simulink model "Lab2_Task_5_advanced"  (R2025b)
settings: Solver=FixedStepAuto  StartTime=0.0  StopTime=inf  RelTol=1e-3
model workspace (MAT data in the model file):
  SL_ROS_VariableLengthArrays_MaxSizes : object (value not decoded)
undefined symbols (not defined in the file or in its folder): angdiff, header, twist
libraries: ros2lib x4, simulink_extras x1, simulink x1
(part 2 of 2)

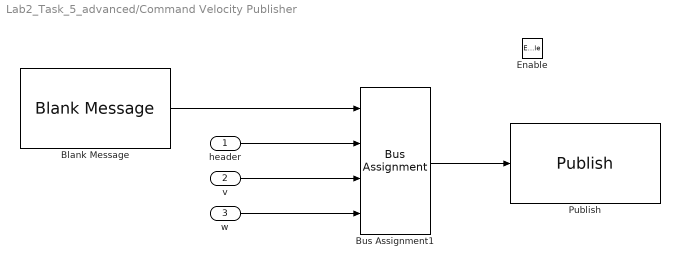
== system Lab2_Task_5_advanced/Command Velocity Publisher ==
  header : Inport
  v : Inport  Port=2
  w : Inport  Port=3
  Enable : EnablePort
  Blank Message : ros2lib/Blank Message  messageClass=Message  entityType=geometry_msgs/TwistStamped  messageType=geometry_msgs/TwistStamped  SampleTime=inf
  Bus Assignment1 : BusAssignment  DialogController=Simulink.DDGSource_BusAssignment  AssignedSignals=header,twist.linear.x,twist.angular.z
  Publish : ros2lib/Publish  topicSource=Select from ROS network  topic=/cmd_vel  messageType=geometry_msgs/TwistStamped  QOSHistory=Keep last  QOSDepth=10  QOSReliability=Reliable  QOSDurability=Volatile  QOSDeadline=Inf  QOSLifespan=Inf  QOSLiveliness=Automatic  QOSLeaseDuration=Inf  QOSAvoidROSNamespaceConventions=off
  wires:
  Bus Assignment1/1 -> Publish/1
  Blank Message/1 -> Bus Assignment1/1
  header/1 -> Bus Assignment1/2
  v/1 -> Bus Assignment1/3
  w/1 -> Bus Assignment1/4

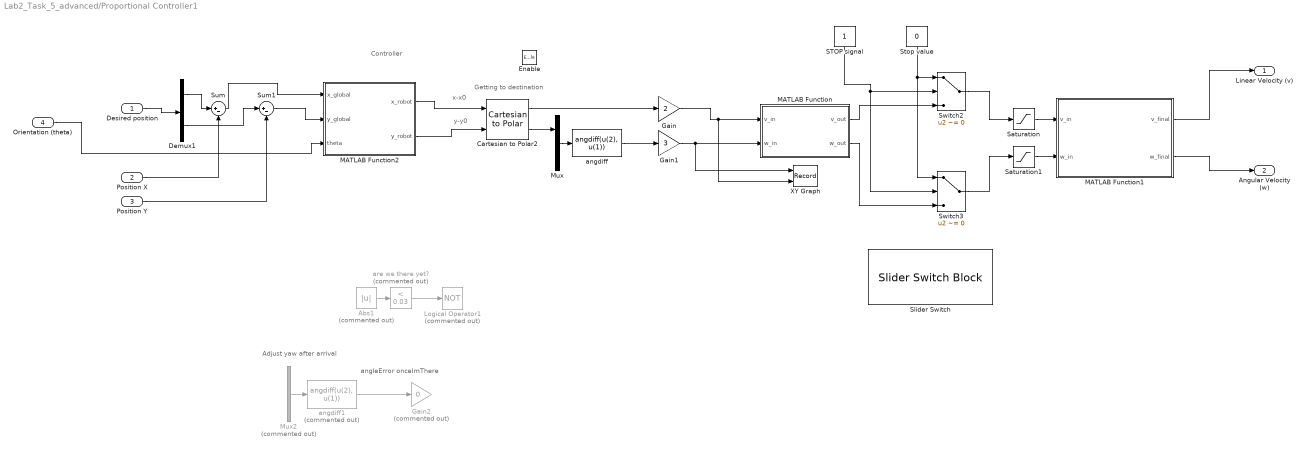
== system Lab2_Task_5_advanced/Proportional Controller1 ==
  note: angleError
      | onceImThere
  note: Controller
  note: x-x0
  note: y-y0
  note: Adjust yaw after arrival
  note: Getting to destination
  Desired position : Inport
  Position X : Inport  Port=2
  Position Y : Inport  Port=3
  Orientation (theta) : Inport  Port=4
  Enable : EnablePort
  Abs1 : Abs  Commented=on  SaturateOnIntegerOverflow=off
  Cartesian to Polar2 : simulink_extras/Transformations/Cartesian to Polar
  Demux1 : Demux  Outputs=2
  Gain : Gain  Gain=2
  Gain1 : Gain  Gain=3
  Gain2 : Gain  Commented=on  Gain=0
  Logical Operator1 : Logic  Commented=on  Operator=NOT  AllPortsSameDT=off  OutDataTypeStr=boolean
  MATLAB Function : MATLAB Function  TreatAsAtomicUnit=on
  MATLAB Function1 : MATLAB Function  TreatAsAtomicUnit=on
  MATLAB Function2 : MATLAB Function  TreatAsAtomicUnit=on
  Mux : Mux  Inputs=2
  Mux2 : Mux  Commented=on  Inputs=2
  "STOP signal " : Constant
  Saturation : Saturate  UpperLimit=0.3  LowerLimit=-0.3  LinearizeAsGain=off
  Saturation1 : Saturate  UpperLimit=999  LowerLimit=-999  LinearizeAsGain=off
  Slider Switch : SliderSwitchBlock
  Stop value : Constant  Value=0
  Sum : Sum  Inputs=|+-
  Sum1 : Sum  Inputs=|+-
  Switch2 : Switch  Criteria=u2 ~= 0  SaturateOnIntegerOverflow=off  InputSameDT=off
  Switch3 : Switch  Criteria=u2 ~= 0  SaturateOnIntegerOverflow=off  InputSameDT=off
  XY Graph : Record  NumPorts=2.0  FileSettingsInternal="{\"entries\":[{\"content\":{\"excelSettings\":{\"content\":{},\"type\":\"Streamout.ExcelSettings\"},\"parquetSettings\":{\"content\":{},\"type\":\"Streamout.ParquetSettings\"}},\"type\":\"Streamout.FileSettingStorage\",\"uuid\":\"\"}],\"packageUris\":[\"http:\\/\\/schema.mathworks.com\\/mf0\\/streamout_blocks\\/R2020a\"],\"version\":\"1.0\"}"  FrameSettings=[0, 0]  Layout=[1 1]  SignalsInternal="{\"entries\":[{\"content\":{\"signals\":[{\"content\":{\"blockPath\":[],\"dimensions\":[1],\"domain\":\"\",\"lineColor\":\"#139fff\",\"lineWidth\":2,\"port\":1,\"sid\":[\"\"],\"signalID\":1,\"signalName\":\"Gain1\"},\"type\":\"RecordBlkView.Signal\",\"uuid\":\"\"},{\"content\":{\"blockPath\":[],\"dimensions\":[1],\"domain\":\"\",\"lineColor\":\"#ff6929\",\"lineWidth\":2,\"port\":2,\"sid\":[\"\"],\"signalID\":2,\"signalName\":\"Gain\"},\"type\":\"RecordBlkView.Signal\",\"uuid\":\"\"}]},\"type\":\"RecordBlkView.InputSignals\",\"uuid\":\"\"}],\"packageUris\":[\"http:\\/\\/schema.mathworks.com\\/mf0\\/streamout_blocks\\/R2020a\"],\"version\":\"1.0\"}"  VisualizationBindings="{\"xyplotplugin\":{\"info\":[{\"series\":[],\"subplotID\":1}]}}"  CompatibilityTag=XY
  angdiff : MATLABFcn  MATLABFcn=angdiff(u(2), u(1))  OutputDimensions=1  Output1D=off
  angdiff1 : MATLABFcn  Commented=on  MATLABFcn=angdiff(u(2), u(1))  OutputDimensions=1  Output1D=off
  are we there yet? : simulink/Logic and Bit Operations/Compare To Constant  Commented=on  relop=<  const=0.03  OutDataTypeStr=boolean
  Linear Velocity (v) : Outport  VectorParamsAs1DForOutWhenUnconnected=off
  Angular Velocity (w) : Outport  Port=2  VectorParamsAs1DForOutWhenUnconnected=off
  wires:
  Mux/1 -> angdiff/1
  Demux1/1 -> Sum/1
  Gain1/1 -> MATLAB Function/2(w_in), XY Graph/1
  "STOP signal "/1 -> Switch2/2, Switch3/2
  Switch3/1 -> Saturation1/1
  Demux1/2 -> Sum1/1
  Cartesian to Polar2/2 -> Mux/1
  Stop value/1 -> Switch2/1, Switch3/1
  Desired position/1 -> Demux1/1
  Orientation (theta)/1 -> MATLAB Function2/3(theta)
  Position X/1 -> Sum/2
  Position Y/1 -> Sum1/2
  Saturation1/1 -> MATLAB Function1/2(w_in)
  angdiff1/1 -> Gain2/1
  Saturation/1 -> MATLAB Function1/1(v_in)
  Sum1/1 -> MATLAB Function2/2(y_global)
  Abs1/1 -> are we there yet?/1
  Cartesian to Polar2/1 -> Gain/1
  angdiff/1 -> Gain1/1
  Sum/1 -> MATLAB Function2/1(x_global)
  Switch2/1 -> Saturation/1
  are we there yet?/1 -> Logical Operator1/1
  Mux2/1 -> angdiff1/1
  Gain/1 -> XY Graph/2, MATLAB Function/1(v_in)
  MATLAB Function/1(v_out) -> Switch2/3
  MATLAB Function/2(w_out) -> Switch3/3
  MATLAB Function1/1(v_final) -> Linear Velocity (v)/1
  MATLAB Function1/2(w_final) -> Angular Velocity (w)/1
  MATLAB Function2/1(x_robot) -> Cartesian to Polar2/1
  MATLAB Function2/2(y_robot) -> Cartesian to Polar2/2

== matlab function Lab2_Task_5_advanced/MATLAB Function ==
  data: qx input; theta output; qy input; qz input; qw input
function theta = Quat2Yaw(qx, qy, qz, qw)
%#codegen
% Inputs are quaternion components from /odom:
% orientation.x = qx, .y = qy, .z = qz, .w = qw

% Build 1x4 quaternion row in the order [w x y z]
q = [qw, qx, qy, qz];

% Convert to Euler angles [yaw pitch roll] (ZYX convention)
eul = quat2eul(q, 'ZYX');

% Use yaw (rotation about Z-axis)
theta = eul(1);
end

== matlab function Lab2_Task_5_advanced/MATLAB Function1 ==
  data: ranges input; angle_min input; angle_inc input; pose_x input; pose_y input; pose_theta input; angular_vel input
function PointCloudMapper(ranges, angle_min, angle_inc, pose_x, pose_y, pose_theta, angular_vel)
    %#codegen
    
    % Persistent storage för point cloud och robot trail
    persistent cloud_x cloud_y
    persistent trail_x trail_y
    persistent update_count
    persistent last_plot_time
    
    % Initialisering
    if isempty(cloud_x)
        cloud_x = zeros(100000, 1);
        cloud_y = zeros(100000, 1);
        trail_x = zeros(5000, 1);
        trail_y = zeros(5000, 1);
        update_count = uint32(0);
        last_plot_time = 0;
    end
    
    % Skippa om roboten snurrar för snabbt (förhindrar ghost points)
    if abs(angular_vel) > 0.6
        return;
    end
    
    update_count = update_count + 1;
    
    % --- LIDAR TRANSFORMATION ---
    ranges = double(ranges(:));
    N = length(ranges);
    
    % Beräkna vinklar
    angles = double(angle_min) + (0:N-1)' * double(angle_inc);
    
    % Filtrera giltiga punkter
    valid = isfinite(ranges) & (ranges > 0.12) & (ranges < 3.5);
    
    if sum(valid) < 5
        return; % För få punkter
    end
    
    valid_ranges = ranges(valid);
    valid_angles = angles(valid);
    
    % Konvertera till robot frame (polar -> cartesian)
    robot_x = valid_ranges .* cos(valid_angles);
    robot_y = valid_ranges .* sin(valid_angles);
    
    % Transformera till world frame
    cos_theta = cos(pose_theta);
    sin_theta = sin(pose_theta);
    
    world_x = pose_x + robot_x * cos_theta - robot_y * sin_theta;
    world_y = pose_y + robot_x * sin_theta + robot_y * cos_theta;
    
    % Lägg till punkter i cloud (circular buffer)
    n_new = length(world_x);
    start_idx = mod(double(update_count) * 200, 100000) + 1;
    end_idx = min(start_idx + n_new - 1, 100000);
    actual_n = end_idx - start_idx + 1;
    
    cloud_x(start_idx:end_idx) = world_x(1:actual_n);
    cloud_y(start_idx:end_idx) = world_y(1:actual_n);
    
    % Lägg till robot position i trail
    trail_idx = mod(double(update_count), 5000) + 1;
    trail_x(trail_idx) = pose_x;
    trail_y(trail_idx) = pose_y;
    
    % --- PLOTTING ---
    % Plotta var 15:e uppdatering för bättre performance
    current_time = double(update_count);
    if (current_time - last_plot_time) >= 15
        last_plot_time = current_time;
        
        % Skapa/uppdatera figure
        fig = figure(99);
        clf(fig);
        hold on;
        
        % Plotta LIDAR points (blå, små, transparent)
        valid_cloud = (cloud_x ~= 0) | (cloud_y ~= 0);
        if sum(valid_cloud) > 0
            scatter(cloud_x(valid_cloud), cloud_y(valid_cloud), 1, 'b.', ...
                'MarkerEdgeAlpha', 0.3);
        end
        
        % Plotta robot trajectory (röd linje)
        valid_trail = (trail_x ~= 0) | (trail_y ~= 0);
        if sum(valid_trail) > 1
            plot(trail_x(valid_trail), trail_y(valid_trail), 'r-', 'LineWidth', 2);
        end
        
        % Markera start (gul) och slut (blå)
        trail_indices = find(valid_trail);
        if ~isempty(trail_indices)
            start_idx_trail = trail_indices(1);
            end_idx_trail = trail_indices(end);
            
            plot(trail_x(start_idx_trail), trail_y(start_idx_trail), 'yo', ...
                'MarkerSize', 8, 'MarkerFaceColor', 'y');
            plot(trail_x(end_idx_trail), trail_y(end_idx_trail), 'bo', ...
                'MarkerSize', 8, 'MarkerFaceColor', 'b');
        end
        
        % Formatering
        axis equal;
        grid on;
        xlabel('X (cm)');
        ylabel('Y (cm)');
        title('Following a wall');
        
        % Legend
        legend({'', 'Robots trajectory', 'Start', 'End'}, 'Location', 'best');
        
        % Invertera Y-axeln för att matcha din väns plot
        set(gca, 'YDir', 'reverse');
        
        drawnow limitrate;
    end
end

== matlab function Lab2_Task_5_advanced/carrot_method ==
  data: pose_x input; pose_y input; pose_theta input; ranges input; target_x output; angle_min input; angle_inc input; target_y output
function [target_x, target_y] = FindWallTarget(pose_x, pose_y, pose_theta, ranges, angle_min, angle_inc)
    %#codegen
    
    % --- CONFIGURATION ---
    target_dist = 1.0;   % Target distance from wall (reduced for safety)
    lookahead   = 0.6;   % Forward "Carrot" distance (reduced for stability)
    
    % LIDAR validity constants
    MIN_VALID_RANGE = 0.12;  % TurtleBot3 minimum range
    MAX_VALID_RANGE = 3.5;   % TurtleBot3 maximum range
    MIN_POINTS_NEEDED = 3;   % Minimum points to trust wall detection
    
    % --- DEBUG PRINT ---
    persistent k
    if isempty(k), k = uint32(0); end
    k = k + 1;
    doPrint = (mod(k, uint32(10)) == 0);
    
    % === LIDAR HEALTH CHECK ===
    if doPrint
        ranges_double = double(ranges(:));
        fprintf('=== LIDAR CHECK ===\n');
        fprintf('angle_min: %.3f rad (%.1f deg)\n', angle_min, angle_min*180/pi);
        fprintf('angle_inc: %.5f rad (%.2f deg)\n', angle_inc, angle_inc*180/pi);
        fprintf('Total ranges: %d\n', int32(length(ranges_double)));
        fprintf('Finite ranges: %d\n', int32(sum(isfinite(ranges_double))));
        fprintf('Ranges > 0: %d\n', int32(sum(ranges_double > 0)));
        
        valid_for_debug = isfinite(ranges_double) & (ranges_double >= MIN_VALID_RANGE) & (ranges_double <= MAX_VALID_RANGE);
        if sum(valid_for_debug) > 0
            fprintf('Valid ranges (%.2f-%.2f m): %d\n', MIN_VALID_RANGE, MAX_VALID_RANGE, int32(sum(valid_for_debug)));
            fprintf('Min dist: %.3fm\n', min(ranges_double(valid_for_debug)));
            fprintf('Max dist: %.3fm\n', max(ranges_double(valid_for_debug)));
            fprintf('Mean dist: %.3fm\n', mean(ranges_double(valid_for_debug)));
        else
            fprintf('*** WARNING: NO VALID LIDAR DATA! ***\n');
        end
        fprintf('==================\n');
    end
    
    % --- 1. DATA PREP ---
    ranges = double(ranges(:));
    N = length(ranges);
    raw_angles = double(angle_min) + (0:N-1)' * double(angle_inc);
    angles = mod(raw_angles + pi, 2*pi) - pi;
    
    % --- 2. FIND WALL (RIGHT SIDE WITH EXPANDED SEARCH) ---
    % Primary search: -120° to -40° (right rear to right front)
    search_min = -120 * (pi/180);
    search_max = -40  * (pi/180);
    mask = (angles >= search_min) & (angles <= search_max);
    
    % Apply strict validity filter
    valid_mask = isfinite(ranges) & (ranges >= MIN_VALID_RANGE) & (ranges <= MAX_VALID_RANGE);
    combined_mask = mask & valid_mask;
    
    valid_r = ranges(combined_mask);
    valid_a = angles(combined_mask);
    
    % === CRITICAL: Check if we have enough points ===
    if length(valid_r) < MIN_POINTS_NEEDED
        if doPrint
            fprintf('INSUFFICIENT WALL DATA (%d points) - Expanding Search\n', int32(length(valid_r)));
        end
        
        % Fallback 1: Expand to full right side (-180° to 0°)
        search_min = -180 * (pi/180);
        search_max = 0 * (pi/180);
        mask = (angles >= search_min) & (angles <= search_max);
        combined_mask = mask & valid_mask;
        
        valid_r = ranges(combined_mask);
        valid_a = angles(combined_mask);
        
        if length(valid_r) < MIN_POINTS_NEEDED
            % Fallback 2: EMERGENCY - No wall found, execute recovery behavior
            if doPrint
                fprintf('WALL COMPLETELY LOST - RECOVERY MODE\n');
            end
            
            % Recovery: Move forward-left to search for wall
            local_x = 0.2;  % Slow forward
            local_y = 0.15; % Drift left to find wall
            
            % Transform to global and return
            global_x_rel = local_x * cos(pose_theta) - local_y * sin(pose_theta);
            global_y_rel = local_x * sin(pose_theta) + local_y * cos(pose_theta);
            target_x = pose_x + global_x_rel;
            target_y = pose_y + global_y_rel;
            return;
        end
    end
    
    % --- 3. WALL PROCESSING ---
    % Find closest point (with safety check)
    [d_curr, idx] = min(valid_r);
    
    % Safety: Clamp distance to reasonable range
    d_curr = max(MIN_VALID_RANGE, min(d_curr, MAX_VALID_RANGE));
    
    % Stabilize Angle (Average nearby points with bounds checking)
    w = 2;
    i_start = max(1, idx - w);
    i_end   = min(length(valid_a), idx + w);
    
    % Additional safety: ensure we have points to average
    if i_start <= i_end
        alpha = mean(valid_a(i_start:i_end));
    else
        alpha = valid_a(idx);  % Fallback to single point
    end
    
    % --- 4. GEOMETRY ---
    % Normal (Wall -> Robot, pointing AWAY from wall)
    nx = -cos(alpha);
    ny = -sin(alpha);
    
    % Tangent (Forward along right wall)
    tx = ny;
    ty = -nx;
    
    % Error from target distance
    err = d_curr - target_dist;
    
    % CARROT CALCULATION (with error correction)
    local_x = (lookahead * tx) - (err * nx);
    local_y = (lookahead * ty) - (err * ny);
    
    if doPrint
        fprintf('WALL FOUND: d=%.2fm err=%.2fm ang=%.1f° pts=%d | Carrot: [%.2f, %.2f]\n', ...
            d_curr, err, alpha*180/pi, int32(length(valid_r)), local_x, local_y);
    end
    
    % --- 5. GLOBAL TRANSFORM ---
    global_x_rel = local_x * cos(pose_theta) - local_y * sin(pose_theta);
    global_y_rel = local_x * sin(pose_theta) + local_y * cos(pose_theta);
    
    target_x = pose_x + global_x_rel;
    target_y = pose_y + global_y_rel;
end

== matlab function Lab2_Task_5_advanced/Proportional Controller1/MATLAB Function ==
  data: v_in input; v_out output; w_in input; w_out output
function [v_out, w_out] = velocity_monitor(v_in, w_in)
    %#codegen
    persistent counter
    if isempty(counter), counter = uint32(0); end
    counter = counter + 1;
    
    if mod(counter, uint32(5)) == 0
        fprintf('>>> SENDING TO ROBOT: v=%.4f m/s, w=%.4f rad/s\n', v_in, w_in);
    end
    
    v_out = v_in;
    w_out = w_in;
end

== matlab function Lab2_Task_5_advanced/Proportional Controller1/MATLAB Function1 ==
  data: v_in input; v_final output; w_in input; w_final output
function [v_final, w_final] = final_debug(v_in, w_in)
    %#codegen
    persistent counter
    if isempty(counter), counter = uint32(0); end
    counter = counter + 1;
    
    if mod(counter, uint32(5)) == 0
        fprintf('>>> SENDING TO ROBOT: v=%.4f m/s, w=%.4f rad/s\n', v_in, w_in);
    end
    
    v_final = v_in;
    w_final = w_in;
end

== matlab function Lab2_Task_5_advanced/MATLAB Function3 ==
  data: L input; xv output; yv output
function [xv, yv] = fcn(L)
%#codegen

a = L(1);
b = L(2);
c = L(3);


% ====== inställningar (ändra vid behov) ======
N    = 20;     % antal punkter (FAST)
xmin = -2; xmax = 2;
ymin = -2; ymax = 2;
epsb = 1e-9;

% ====== skapa x-grid en gång ======
persistent xgrid ygrid
if isempty(xgrid)
    xgrid = linspace(xmin, xmax, N)';   % Nx1
    ygrid = zeros(N,1);                 % Nx1
end

if abs(b) > epsb
    % ax + by + c = 0  =>  y = (-a*x - c)/b
    xv = xgrid;
    yv = (-a.*xgrid - c) ./ b;
else
    % vertikal linje: ax + c = 0 => x = -c/a
    xv = (-c./a) * ones(N,1);
    yv = linspace(ymin, ymax, N)';      % Nx1
end

== matlab function Lab2_Task_5_advanced/Proportional Controller1/MATLAB Function2 ==
  data: x_global input; x_robot output; y_robot output; y_global input; theta input
function [x_robot, y_robot] = global_to_robot(x_global, y_global, theta)
    %#codegen
    % Transform global error to robot frame
    x_robot = x_global * cos(theta) + y_global * sin(theta);
    y_robot = -x_global * sin(theta) + y_global * cos(theta);
end
